simulink model "Controller"  (R2025b)
settings: Solver=VariableStepAuto  StartTime=0.0  StopTime=10.0  RelTol=1e-3
settings Model: Creator=Ishwar  LastModifiedBy=Ishwar

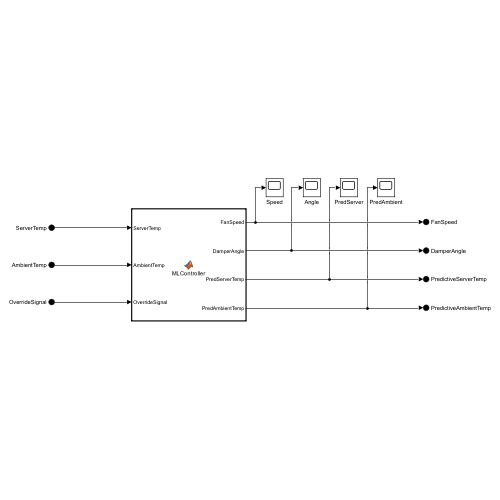
[thumbnail: Simulink's stored preview of the top-level diagram]
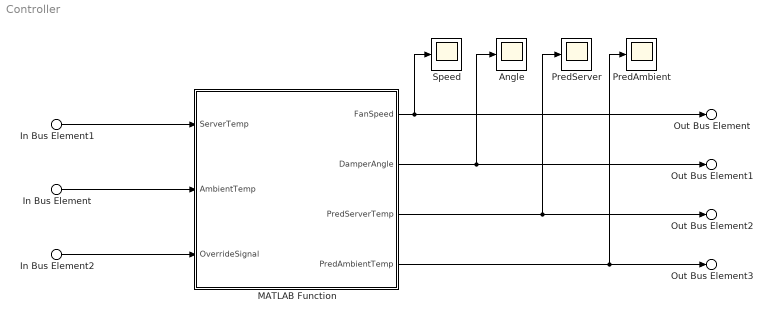
== system Controller ==
  In Bus Element : Inport  PortName=AmbientTemp
  In Bus Element1 : Inport  Port=2  PortName=ServerTemp
  In Bus Element2 : Inport  Port=3  PortName=OverrideSignal
  Angle : Scope
      settings: ActiveDisplayYMinimum=-43.4706757513296  ActiveDisplayYMaximum=88.371478876228139
  MATLAB Function : MATLAB Function  TreatAsAtomicUnit=on
  PredAmbient : Scope
      settings: DataLoggingVariableName=ScopeData2
  PredServer : Scope
      settings: DataLoggingVariableName=ScopeData3
  Speed : Scope
      settings: ActiveDisplayYMinimum=-66.4281757157633  ActiveDisplayYMaximum=80.169630565365139
  Out Bus Element : Outport  PortName=FanSpeed
  Out Bus Element1 : Outport  Port=2  PortName=DamperAngle
  Out Bus Element2 : Outport  Port=3  PortName=PredictiveServerTemp
  Out Bus Element3 : Outport  Port=4  PortName=PredictiveAmbientTemp
  wires:
  MATLAB Function/2(DamperAngle) -> Out Bus Element1/1, Angle/1
  In Bus Element/1 -> MATLAB Function/2(AmbientTemp)
  In Bus Element1/1 -> MATLAB Function/1(ServerTemp)
  MATLAB Function/1(FanSpeed) -> Out Bus Element/1, Speed/1
  In Bus Element2/1 -> MATLAB Function/3(OverrideSignal)
  MATLAB Function/4(PredAmbientTemp) -> Out Bus Element3/1, PredAmbient/1
  MATLAB Function/3(PredServerTemp) -> Out Bus Element2/1, PredServer/1

== matlab function Controller/MATLAB Function ==
  data: ServerTemp input; FanSpeed output; AmbientTemp input; DamperAngle output; PredServerTemp output; PredAmbientTemp output; OverrideSignal input
function [FanSpeed, DamperAngle, PredServerTemp, PredAmbientTemp] = MLController(ServerTemp, AmbientTemp, OverrideSignal)
%#codegen
% Inputs:
%   ServerTemp, AmbientTemp - sensor temperatures
%   OverrideSignal          - 0 (normal) or non-zero (variation mode)
% Outputs:
%   FanSpeed, DamperAngle   - actuator commands
%   PredServerTemp, PredAmbientTemp - predictive temperatures

% --- Persistent model handles ---
persistent mdlFan mdlDamper mdlPredServer mdlPredAmbient
if isempty(mdlFan)
    mdlFan = loadLearnerForCoder('FanSpeedModel');
end
if isempty(mdlDamper)
    mdlDamper = loadLearnerForCoder('DamperAngleModel');
end
if isempty(mdlPredServer)
    mdlPredServer = loadLearnerForCoder('PredServerTempModel');
end
if isempty(mdlPredAmbient)
    mdlPredAmbient = loadLearnerForCoder('PredAmbientTempModel');
end

% --- Predictions ---
FanSpeed        = predict(mdlFan, [ServerTemp, AmbientTemp]);
DamperAngle     = predict(mdlDamper, [ServerTemp, AmbientTemp]);
PredServerTemp  = predict(mdlPredServer, [ServerTemp, AmbientTemp]);
PredAmbientTemp = predict(mdlPredAmbient, [ServerTemp, AmbientTemp]);

% --- Override logic ---
if OverrideSignal ~= 0
    % Apply ±2 random variation when override is non-zero
    FanSpeed    = FanSpeed    + (rand()*4 - 2); % jitter between -2 and +2
    DamperAngle = DamperAngle + (rand()*4 - 2);
end

% --- Saturation ---
FanSpeed    = max(0, min(100, FanSpeed));   % keep within 0–100%
DamperAngle = max(0, min(75, DamperAngle)); % keep within 0–90 deg

end
